simulink model "Lab3_BreakLight_replacement"  (R2026b)
settings: Solver=FixedStepAuto  StopTime=10  EnableMultiTasking=on
PreLoadFcn:
  | vehicle_data;
undefined symbols (not defined in the file or in its folder): DiscIntNeverNeededParam, magnitude, veh1, veh2, veh3
libraries: simulink x3, sldvlib x1
settings Model: DVDesignModelName=Lab3_BreakLight  STM32="{\"AnalogInput\":[{\"ID\":\"ELEC49X_Vehicle_Model:530\"},{\"ID\":\"1302\"}],\"CANWrite\":[{\"ID\":\"ELEC49X_Vehicle_Model:534\"},{\"ID\":\"ELEC49X_Vehicle_Model:535\"},{\"ID\":\"1311\"},{\"ID\":\"1312\"}],\"DigitalPortRead\":[{\"ID\":\"ELEC49X_Vehicle_Model:563\"},{\"ID\":\"ELEC49X_Vehicle_Model:564\"},{\"ID\":\"ELEC49X_Vehicle_Model:565\"},{\"ID\":\"ELEC49X_Vehicle_Model:566\"},{\"ID\":\"ELEC49X_Vehicle_Model:567\"},{\"ID\":\"ELEC49X_Vehicle_Model:589\"},{\"ID\":\"ELEC49X_Vehicle_Model:1023\"},{\"ID\":\"1368\"},{\"ID\":\"1369\"},{\"ID\":\"1370\"},{\"ID\":\"1371\"},{\"ID\":\"1372\"},{\"ID\":\"1401\"},{\"ID\":\"1402\"}],\"SPIControllerTransmit\":[{\"ID\":\"ELEC49X_Vehicle_Model:953\"},{\"ID\":\"1404\"}],\"SPIControllerReceive\":[{\"ID\":\"ELEC49X_Vehicle_Model:1097\"},{\"ID\":\"1403\"}]}"  Creator=jckwe  LastModifiedBy=balog
settings OptimizationCC: DefaultParameterBehavior=Inlined  DifferentSizesBufferReuse=on  EfficientTunableParamExpr=on  EnhancedBackFolding=on  MaxStackSize=64  OptimizationCustomize=off  OptimizeBlockOrder=speed  PassReuseOutputArgsAs=Individual arguments  RemoveInternalMemoryZeroInit=on  RemoveRootLevelIOMemoryZeroInit=on
settings DebuggingCC: ParameterTunabilityLossMsg=error  SaveWithDisabledLinksMsg=none  SaveWithParameterizedLinksMsg=none
settings HardwareCC: ProdHWDeviceType=ARM Compatible->ARM Cortex-M  ProdLargestAtomicFloat=Double  ProdLargestAtomicInteger=Long  ProdLongLongMode=on
settings SFSimCC: MATLABDynamicMemAlloc=off
settings RTWCC: BuildConfiguration=Faster Runs  Description=Embedded Coder  GPUComputeCapability=5.0  GenerateReport=on  HardwareBoard=STM32F4xx Based  SystemTargetFile=ert.tlc  TLCOptions=-aInlineSetEventsForThisBaseRateFcn=TLC_FALSE -aSuppressMultiTaskScheduler=TLC_FALSE -aRateBasedStepFcn=1  TemplateMakefile=ert_default_tmf
settings CodeAppCC: ForceParamTrailComments=on  IgnoreCustomStorageClasses=off  InsertBlockDesc=on  OperatorAnnotations=on  SFDataObjDesc=on  SimulinkDataObjDesc=on
settings ERTTargetCC: CodeReplacementLibrary=ARM Cortex-M  ExtModeIntrfLevel=Level2 - Open  ExtModeMexFile=ext_xcp  ExtModeStaticAlloc=on  SupportContinuousTime=on
settings ConfigComp: DVCodeAnalysisIgnoreVolatile=off  DVDefectChecker=on  DVDetectOutOfBounds=on  DVHarnessSource=Signal Editor  DVModelCoverageObjectives=MCDC  DVModelReferenceHarness=on  DVParametersConfigFileName=vehicle_data.m  DVSFcnSupport=off  DVTestSuiteOptimization=Auto

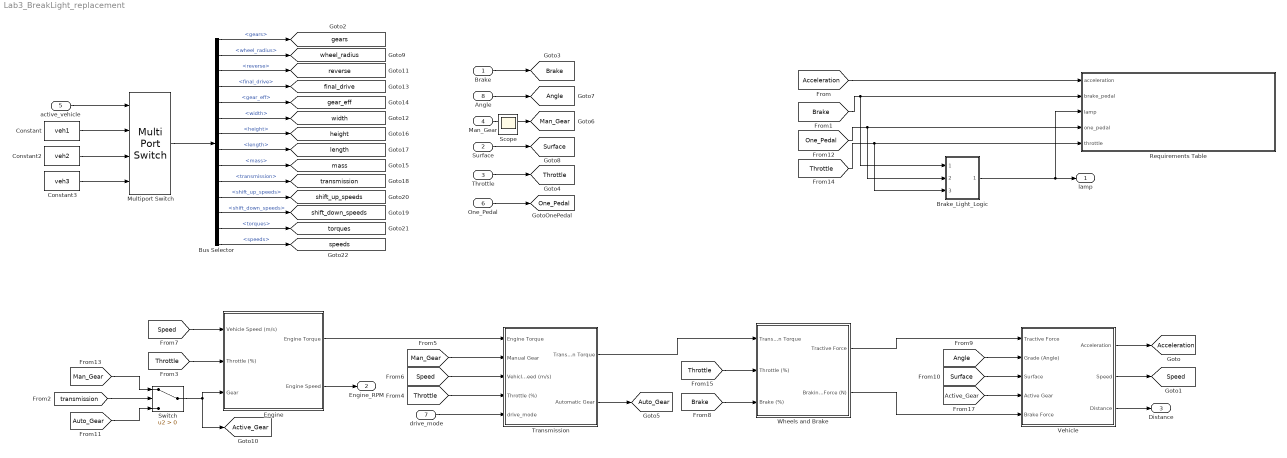
== system Lab3_BreakLight_replacement ==
  Brake : Inport
  Surface : Inport  Port=2
  Throttle : Inport  Port=3  OutMin=0  OutMax=100  OutDataTypeStr=double  LockScale=on
  Man_Gear : Inport  Port=4  OutDataTypeStr=int8
  active_vehicle : Inport  Port=5  OutMin=1  OutMax=3
  One_Pedal : Inport  Port=6  OutMin=0  OutDataTypeStr=int8
  drive_mode : Inport  Port=7  OutMin=-1  OutMax=3  OutDataTypeStr=int8
  Angle : Inport  Port=8
  Brake_Light_Logic : Subsystem
  Bus Selector : BusSelector  OutputSignals=gears,wheel_radius,reverse,final_drive,gear_eff,width,height,length,mass,transmission,shift_up_speeds,shift_down_speeds,torques,speeds
  Constant : Constant  Value=veh1  OutDataTypeStr=Bus: VehicleBus
  Constant2 : Constant  Value=veh2  OutDataTypeStr=Bus: VehicleBus
  Constant3 : Constant  Value=veh3  OutDataTypeStr=Bus: VehicleBus
  Engine : Subsystem
      mask Display: image('Engine Icon.png',[40 40 60 60]);
  Multiport Switch : MultiPortSwitch  SaturateOnIntegerOverflow=off  InputSameDT=off
  Requirements Table : Requirements Table  TreatAsAtomicUnit=on
  Switch : Switch  Criteria=u2 > Threshold  SaturateOnIntegerOverflow=off  InputSameDT=off
  Transmission : Subsystem
      mask Display: image('Transmission Icon.png', [40 40 60 60]);
  Vehicle : Subsystem
      mask Display: image('Vehicle Icon.png', [40 40 60 60]);
  Wheels and Brake : Subsystem
      mask Display: image('Wheel Icon.png', [40 40 60 60]);
  lamp : Outport
  Engine_RPM : Outport  Port=2
  Distance : Outport  Port=3
  Scope : Scope
  tag scope: Acceleration=global, Active_Gear=global, Angle=global, Auto_Gear=global, Brake=global, Man_Gear=global, One_Pedal=global, Speed=global, Surface=global, Throttle=global, final_drive=global, gear_eff=global, gears=global, height=global, length=global, mass=global, reverse=global, shift_down_speeds=global, shift_up_speeds=global, speeds=global, torques=global, transmission=global, wheel_radius=global, width=global
  wires:
  Vehicle/3(Distance) -> Distance/1
  Vehicle/2(Speed) -> [Speed]
  Vehicle/1(Acceleration) -> [Acceleration]
  Transmission/1(Transmission Torque) -> Wheels and Brake/1(Transmission Torque)
  Engine/1(Engine Torque) -> Transmission/1(Engine Torque)
  Wheels and Brake/1(Tractive Force) -> Vehicle/1(Tractive Force)
  [Throttle] -> Engine/2(Throttle (%))
  [Throttle] -> Transmission/4(Throttle (%))
  [Speed] -> Transmission/3(Vehicle Speed (m/s))
  [Speed] -> Engine/1(Vehicle Speed (m/s))
  [Brake] -> Wheels and Brake/3(Brake (%))
  [Angle] -> Vehicle/2(Grade (Angle))
  [Surface] -> Vehicle/3(Surface)
  Transmission/2(Automatic Gear) -> [Auto_Gear]
  Engine/2(Engine Speed) -> Engine_RPM/1
  Switch/1 -> [Active_Gear], Engine/3(Gear)
  [transmission] -> Switch/2
  [Man_Gear] -> Switch/1
  [Auto_Gear] -> Switch/3
  [Active_Gear] -> Vehicle/4(Active Gear)
  Wheels and Brake/2(Braking Force (N)) -> Vehicle/5(Brake Force)
  [Throttle] -> Wheels and Brake/2(Throttle (%))
  Brake/1 -> [Brake]
  Angle/1 -> [Angle]
  Man_Gear/1 -> [Man_Gear]
  Surface/1 -> [Surface]
  [Brake] -> Brake_Light_Logic/1(Brake), Requirements Table/2(brake_pedal)
  active_vehicle/1 -> Multiport Switch/1
  Constant/1 -> Multiport Switch/2
  Constant2/1 -> Multiport Switch/3
  Constant3/1 -> Multiport Switch/4
  Multiport Switch/1 -> Bus Selector/1
  Bus Selector/1 -> [gears]  "<gears>"
  Bus Selector/3 -> [reverse]  "<reverse>"
  Bus Selector/2 -> [wheel_radius]  "<wheel_radius>"
  Bus Selector/14 -> [speeds]  "<speeds>"
  Bus Selector/13 -> [torques]  "<torques>"
  Bus Selector/12 -> [shift_down_speeds]  "<shift_down_speeds>"
  Bus Selector/10 -> [transmission]  "<transmission>"
  Bus Selector/9 -> [mass]  "<mass>"
  Bus Selector/11 -> [shift_up_speeds]  "<shift_up_speeds>"
  Bus Selector/8 -> [length]  "<length>"
  Bus Selector/7 -> [height]  "<height>"
  Bus Selector/6 -> [width]  "<width>"
  Bus Selector/5 -> [gear_eff]  "<gear_eff>"
  Bus Selector/4 -> [final_drive]  "<final_drive>"
  Throttle/1 -> [Throttle]
  [Man_Gear] -> Transmission/2(Manual Gear)
  One_Pedal/1 -> [One_Pedal]
  drive_mode/1 -> Transmission/5(drive_mode)
  [Acceleration] -> Requirements Table/1(acceleration)
  [One_Pedal] -> Brake_Light_Logic/2(One_Pedal), Requirements Table/4(one_pedal)
  [Throttle] -> Brake_Light_Logic/3(Throttle), Requirements Table/5(throttle)
  Brake_Light_Logic/1(Out1) -> lamp/1, Requirements Table/3(lamp)

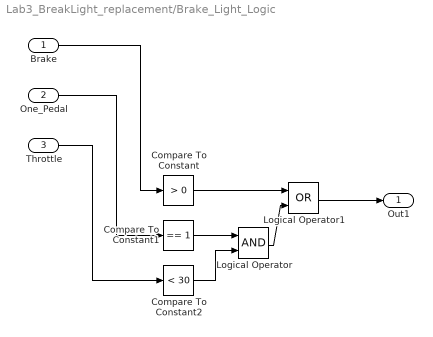
== system Lab3_BreakLight_replacement/Brake_Light_Logic ==
  Brake : Inport
  One_Pedal : Inport  Port=2
  Throttle : Inport  Port=3
  Compare To Constant : simulink/Logic and Bit Operations/Compare To Constant  relop=>  const=0  OutDataTypeStr=boolean
  Compare To Constant1 : simulink/Logic and Bit Operations/Compare To Constant  relop===  const=1  OutDataTypeStr=boolean
  Compare To Constant2 : simulink/Logic and Bit Operations/Compare To Constant  relop=<  const=30  OutDataTypeStr=boolean
  Logical Operator : Logic  AllPortsSameDT=off  OutDataTypeStr=boolean
  Logical Operator1 : Logic  Operator=OR  AllPortsSameDT=off  OutDataTypeStr=boolean
  Out1 : Outport
  wires:
  Logical Operator1/1 -> Out1/1
  Logical Operator/1 -> Logical Operator1/2
  Brake/1 -> Compare To Constant/1
  Throttle/1 -> Compare To Constant2/1
  Compare To Constant2/1 -> Logical Operator/2
  One_Pedal/1 -> Compare To Constant1/1
  Compare To Constant/1 -> Logical Operator1/1
  Compare To Constant1/1 -> Logical Operator/1

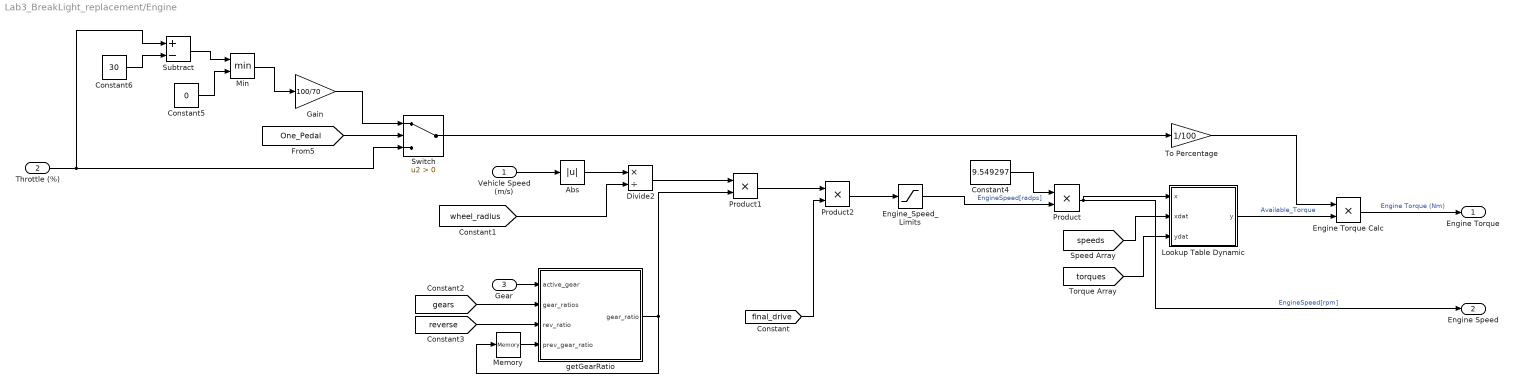
== system Lab3_BreakLight_replacement/Engine ==
  Vehicle Speed (m/s) : Inport
  Throttle (%) : Inport  Port=2
  Gear : Inport  Port=3  OutDataTypeStr=int8
  Abs : Abs  SaturateOnIntegerOverflow=off
  Constant4 : Constant  Value=9.549297
  Constant5 : Constant  Value=0
  Constant6 : Constant  Value=30
  Divide2 : Product  Inputs=*/
  Engine Torque Calc : Product
  Engine_Speed_Limits : Saturate  UpperLimit=800  LowerLimit=80
  Gain : Gain  Gain=100/70
  Lookup Table Dynamic : Subsystem  mask(Sldv Lookup Table Dynamic Replacement){LookUpMeth=Interpolation-Use End Values, OutDataTypeStr=double, LockScale=off, RndMeth=Floor, DoSatur=off}
      mask prompts: LookUpMeth "Lookup Method:"; OutDataTypeStr "Output data type:"; LockScale "Lock output data type setting against changes by the fixed-point tools"; RndMeth "Integer rounding mode:"; DoSatur "Do Saturation"
      mask init:
      | mode = LookUpMeth-1;
      mask TypeOptions LookUpMeth: Interpolation-Extrapolation | Interpolation-Use End Values | Use Input Nearest | Use Input Below | Use Input Above
      mask Callback OutDataTypeStr: fixptdialog(gcbh)
      mask TypeOptions RndMeth: Ceiling | Convergent | Floor | Nearest | Round | Simplest | Zero
  Memory : Memory
  Min : MinMax  Inputs=2
  Product : Product
  Product1 : Product
  Product2 : Product
  Subtract : Sum  Inputs=+-
  Switch : Switch  Criteria=u2 > Threshold  SaturateOnIntegerOverflow=off  InputSameDT=off
  To Percentage : Gain  Gain=1/100
  getGearRatio : MATLAB Function  TreatAsAtomicUnit=on
  Engine Torque : Outport
  Engine Speed : Outport  Port=2
  wires:
  To Percentage/1 -> Engine Torque Calc/1
  Engine_Speed_Limits/1 -> Product/2  "EngineSpeed[radps]"
  Product/1 -> Lookup Table Dynamic/1(x), Engine Speed/1  "EngineSpeed[rpm]"
  [speeds] -> Lookup Table Dynamic/2(xdat)
  [torques] -> Lookup Table Dynamic/3(ydat)
  Engine Torque Calc/1 -> Engine Torque/1  "Engine Torque (Nm)"
  Gear/1 -> getGearRatio/1(active_gear)
  [wheel_radius] -> Divide2/2
  Vehicle Speed (m/s)/1 -> Abs/1
  Divide2/1 -> Product1/1
  getGearRatio/1(gear_ratio) -> Product1/2, Memory/1
  [gears] -> getGearRatio/2(gear_ratios)
  [reverse] -> getGearRatio/3(rev_ratio)
  Memory/1 -> getGearRatio/4(prev_gear_ratio)
  Constant4/1 -> Product/1
  Product1/1 -> Product2/1
  [final_drive] -> Product2/2
  Product2/1 -> Engine_Speed_Limits/1
  Abs/1 -> Divide2/1
  [One_Pedal] -> Switch/2
  Switch/1 -> To Percentage/1
  Throttle (%)/1 -> Subtract/1, Switch/3
  Gain/1 -> Switch/1
  Constant6/1 -> Subtract/2
  Subtract/1 -> Min/1
  Min/1 -> Gain/1
  Constant5/1 -> Min/2
  Lookup Table Dynamic/1(y) -> Engine Torque Calc/2  "Available_Torque"

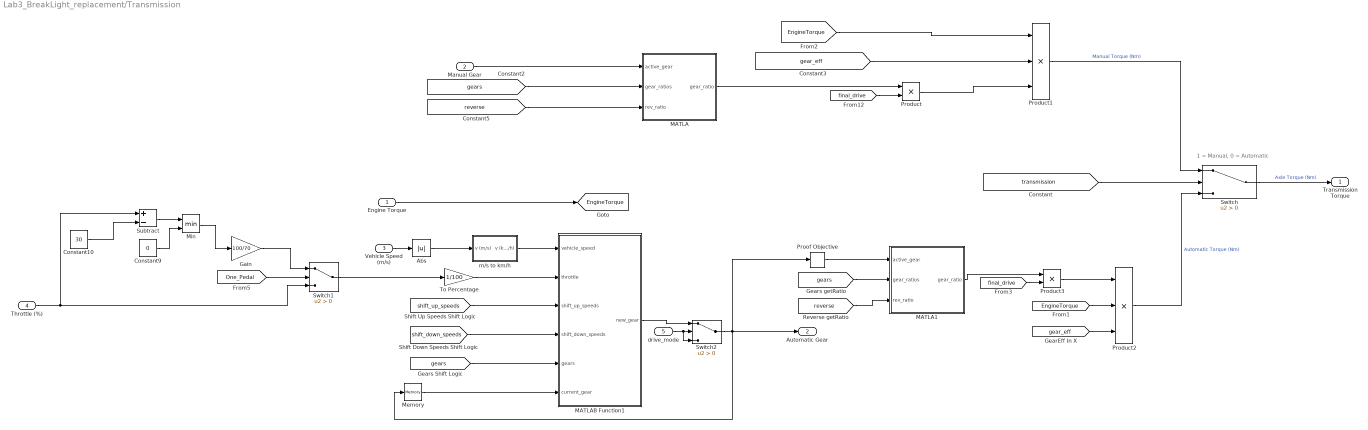
== system Lab3_BreakLight_replacement/Transmission ==
  note: 1 = Manual, 0 = Automatic
  Engine Torque : Inport
  Manual Gear : Inport  Port=2  OutDataTypeStr=int8
  Vehicle Speed (m/s) : Inport  Port=3
  Throttle (%) : Inport  Port=4
  drive_mode : Inport  Port=5  OutMin=-1  OutMax=127  OutDataTypeStr=int8
  Abs : Abs  SaturateOnIntegerOverflow=off
  Constant10 : Constant  Value=30
  Constant9 : Constant  Value=0
  Gain : Gain  Gain=100/70
  MATLA : MATLAB Function  TreatAsAtomicUnit=on
  MATLA1 : MATLAB Function  TreatAsAtomicUnit=on
  MATLAB Function1 : MATLAB Function  TreatAsAtomicUnit=on
  Memory : Memory
  Min : MinMax  Inputs=2
  Product : Product
  Product1 : Product  Inputs=3
  Product2 : Product  Inputs=3
  Product3 : Product
  Proof Objective : sldvlib/Objectives and Constraints/Proof Objective  enabled=on  customAVTBlockType=Proof Objective  intervals={-1, 127}  dispValues=on  outEnabled=on  enableStopSim=off
      settings: AttributesFormatString=%<intervals>
  Subtract : Sum  Inputs=+-
  Switch : Switch  Criteria=u2 > Threshold  SaturateOnIntegerOverflow=off  InputSameDT=off
  Switch1 : Switch  Criteria=u2 > Threshold  SaturateOnIntegerOverflow=off  InputSameDT=off
  Switch2 : Switch  Criteria=u2 > Threshold  SaturateOnIntegerOverflow=off  InputSameDT=off
  To Percentage : Gain  Gain=1/100
  m/s to km/h : Subsystem
  Transmission Torque : Outport
  Automatic Gear : Outport  Port=2
  tag scope: EngineTorque=global
  wires:
  [transmission] -> Switch/2
  MATLA/1(gear_ratio) -> Product/1
  Manual Gear/1 -> MATLA/1(active_gear)
  [gear_eff] -> Product1/2
  Engine Torque/1 -> [EngineTorque]
  [EngineTorque] -> Product1/1
  Product1/1 -> Switch/1  "Manual Torque (Nm)"
  Switch1/1 -> To Percentage/1
  Vehicle Speed (m/s)/1 -> Abs/1
  MATLA1/1(gear_ratio) -> Product3/1
  [EngineTorque] -> Product2/2
  [gear_eff] -> Product2/3
  Product2/1 -> Switch/3  "Automatic Torque (Nm)"
  m/s to km/h/1(v (km/h)) -> MATLAB Function1/1(vehicle_speed)
  Switch/1 -> Transmission Torque/1  "Axle Torque (Nm)"
  [gears] -> MATLA/2(gear_ratios)
  [gears] -> MATLA1/2(gear_ratios)
  [shift_up_speeds] -> MATLAB Function1/3(shift_up_speeds)
  [shift_down_speeds] -> MATLAB Function1/4(shift_down_speeds)
  [gears] -> MATLAB Function1/5(gears)
  Memory/1 -> MATLAB Function1/6(current_gear)
  [reverse] -> MATLA/3(rev_ratio)
  [reverse] -> MATLA1/3(rev_ratio)
  Abs/1 -> m/s to km/h/1(v (m/s))
  To Percentage/1 -> MATLAB Function1/2(throttle)
  Constant9/1 -> Min/2
  Gain/1 -> Switch1/1
  Min/1 -> Gain/1
  [One_Pedal] -> Switch1/2
  Constant10/1 -> Subtract/2
  Throttle (%)/1 -> Subtract/1, Switch1/3
  Subtract/1 -> Min/1
  Proof Objective/1 -> MATLA1/1(active_gear)
  drive_mode/1 -> Switch2/3, Switch2/2
  MATLAB Function1/1(new_gear) -> Switch2/1
  Switch2/1 -> Memory/1, Proof Objective/1, Automatic Gear/1
  [final_drive] -> Product/2
  Product/1 -> Product1/3
  [final_drive] -> Product3/2
  Product3/1 -> Product2/1

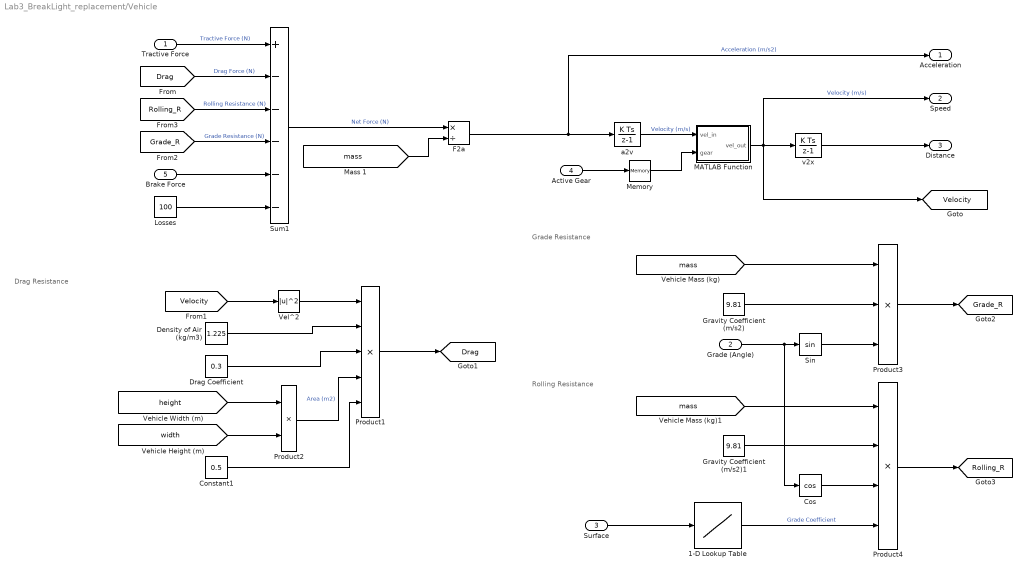
== system Lab3_BreakLight_replacement/Vehicle ==
  note: Rolling Resistance
  note: Grade Resistance
  note: Drag Resistance
  Tractive Force : Inport
  Grade (Angle) : Inport  Port=2
  Surface : Inport  Port=3
  Active Gear : Inport  Port=4
  Brake Force : Inport  Port=5
  1-D Lookup Table : Lookup_n-D  NumberOfTableDimensions=1  BreakpointsForDimension1=[0:4]  Table=[0.015, 0.025, 0.045, 0.09, 0.12]  InternalRulePriority=Speed  RndMeth=Simplest
  Constant1 : Constant  Value=0.5
  Cos : Trigonometry  Operator=cos
  Density of Air (kg/m3) : Constant  Value=1.225
  Drag Coefficient : Constant  Value=0.3
  F2a : Product  Inputs=*/
  Gravity Coefficient (m/s2) : Constant  Value=9.81
  Gravity Coefficient (m/s2)1 : Constant  Value=9.81
  Losses : Constant  Value=100
  MATLAB Function : MATLAB Function  TreatAsAtomicUnit=on
  Memory : Memory
  Product1 : Product  Inputs=5
  Product2 : Product
  Product3 : Product  Inputs=3
  Product4 : Product  Inputs=4
  Sin : Trigonometry
  Sum1 : Sum  Inputs=+-----
  Vel^2 : Math  Operator=magnitude^2  SignedPower=on
  a2v : DiscreteIntegrator  SampleTime=-1  LimitOutput=on  UpperSaturationLimit=100  LowerSaturationLimit=0  ICPrevOutput=DiscIntNeverNeededParam  ICPrevScaledInput=DiscIntNeverNeededParam
  v2x : DiscreteIntegrator  SampleTime=-1  ICPrevOutput=DiscIntNeverNeededParam  ICPrevScaledInput=DiscIntNeverNeededParam
  Acceleration : Outport
  Speed : Outport  Port=2
  Distance : Outport  Port=3
  tag scope: Drag=global, Grade_R=global, Rolling_R=global, Velocity=global
  wires:
  Tractive Force/1 -> Sum1/1  "Tractive Force (N)"
  [Drag] -> Sum1/2  "Drag Force (N)"
  [Rolling_R] -> Sum1/3  "Rolling Resistance (N)"
  [Grade_R] -> Sum1/4  "Grade Resistance (N)"
  Sum1/1 -> F2a/1  "Net Force (N)"
  [mass] -> F2a/2
  [Velocity] -> Vel^2/1
  Vel^2/1 -> Product1/1
  [height] -> Product2/1
  [width] -> Product2/2
  Product2/1 -> Product1/4  "Area (m2)"
  Density of Air (kg/m3)/1 -> Product1/2
  Drag Coefficient/1 -> Product1/3
  Product1/1 -> [Drag]
  [mass] -> Product3/1
  Gravity Coefficient (m/s2)/1 -> Product3/2
  Sin/1 -> Product3/3
  Grade (Angle)/1 -> Cos/1, Sin/1
  Product3/1 -> [Grade_R]
  Cos/1 -> Product4/3
  [mass] -> Product4/1
  Product4/1 -> [Rolling_R]
  Gravity Coefficient (m/s2)1/1 -> Product4/2
  Surface/1 -> 1-D Lookup Table/1
  1-D Lookup Table/1 -> Product4/4  "Grade Coefficient"
  F2a/1 -> Acceleration/1, a2v/1  "Acceleration (m/s2)"
  MATLAB Function/1(vel_out) -> v2x/1, Speed/1, [Velocity]  "Velocity (m/s)"
  Brake Force/1 -> Sum1/5
  Constant1/1 -> Product1/5
  a2v/1 -> MATLAB Function/1(vel_in)  "Velocity (m/s)"
  Active Gear/1 -> Memory/1
  Memory/1 -> MATLAB Function/2(gear)
  Losses/1 -> Sum1/6
  v2x/1 -> Distance/1

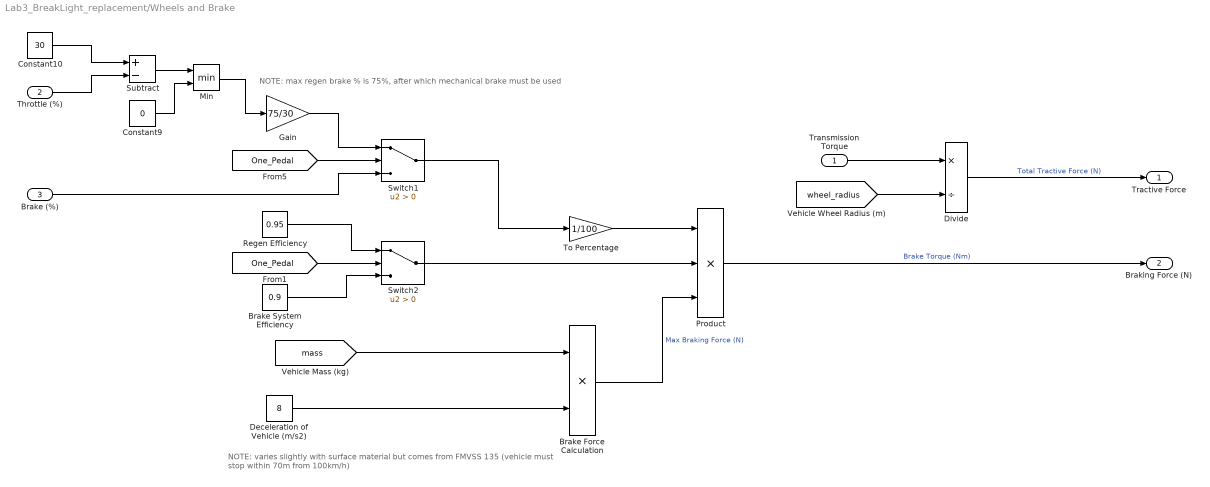
== system Lab3_BreakLight_replacement/Wheels and Brake ==
  note: NOTE: varies slightly with surface material but comes from FMVSS 135 (vehicle
      | must stop within 70m from 100km/h)
  note: NOTE: max regen brake % is 75%, after which mechanical brake must be used
  Transmission Torque : Inport
  Throttle (%) : Inport  Port=2
  Brake (%) : Inport  Port=3
  Brake Force Calculation : Product
  Brake System Efficiency : Constant  Value=0.9
  Constant10 : Constant  Value=30
  Constant9 : Constant  Value=0
  Deceleration of Vehicle (m/s2) : Constant  Value=8
  Divide : Product  Inputs=*/
  Gain : Gain  Gain=75/30
  Min : MinMax  Inputs=2
  Product : Product  Inputs=3
  Regen Efficiency : Constant  Value=0.95
  Subtract : Sum  Inputs=+-
  Switch1 : Switch  Criteria=u2 > Threshold  SaturateOnIntegerOverflow=off  InputSameDT=off
  Switch2 : Switch  Criteria=u2 > Threshold  SaturateOnIntegerOverflow=off  InputSameDT=off
  To Percentage : Gain  Gain=1/100
  Tractive Force : Outport
  Braking Force (N) : Outport  Port=2
  wires:
  Switch2/1 -> Product/2
  Switch1/1 -> To Percentage/1
  Brake Force Calculation/1 -> Product/3  "Max Braking Force (N)"
  Deceleration of Vehicle (m/s2)/1 -> Brake Force Calculation/2
  [mass] -> Brake Force Calculation/1
  Transmission Torque/1 -> Divide/1
  Divide/1 -> Tractive Force/1  "Total Tractive Force (N)"
  To Percentage/1 -> Product/1
  [wheel_radius] -> Divide/2
  Product/1 -> Braking Force (N)/1  "Brake Torque (Nm)"
  Subtract/1 -> Min/1
  Constant9/1 -> Min/2
  Min/1 -> Gain/1
  [One_Pedal] -> Switch1/2
  Gain/1 -> Switch1/1
  Brake (%)/1 -> Switch1/3
  [One_Pedal] -> Switch2/2
  Brake System Efficiency/1 -> Switch2/3
  Regen Efficiency/1 -> Switch2/1
  Constant10/1 -> Subtract/1
  Throttle (%)/1 -> Subtract/2

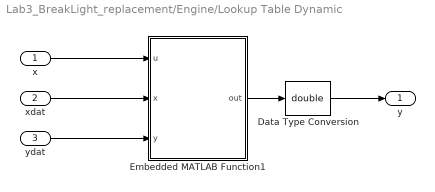
== system Lab3_BreakLight_replacement/Engine/Lookup Table Dynamic ==
  x : Inport  OutDataTypeStr=double  PortDimensions=1
  xdat : Inport  Port=2  OutDataTypeStr=double  PortDimensions=[1 21]
  ydat : Inport  Port=3  OutDataTypeStr=double  PortDimensions=[1 21]
  Data Type Conversion : DataTypeConversion  OutDataTypeStr=double  SaturateOnIntegerOverflow=off  RndMeth=Floor
  Embedded MATLAB Function1 : MATLAB Function  DisableCoverage=on  TreatAsAtomicUnit=on
  y : Outport  OutDataTypeStr=double  PortDimensions=1
  wires:
  Embedded MATLAB Function1/1(out) -> Data Type Conversion/1
  ydat/1 -> Embedded MATLAB Function1/3(y)
  xdat/1 -> Embedded MATLAB Function1/2(x)
  x/1 -> Embedded MATLAB Function1/1(u)
  Data Type Conversion/1 -> y/1

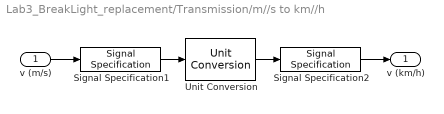
== system Lab3_BreakLight_replacement/Transmission/m//s to km//h ==
  v (m/s) : Inport
  Signal Specification1 : SignalSpecification  Unit=m/s
  Signal Specification2 : SignalSpecification  Unit=km/hr
  Unit Conversion : UnitConversion
  v (km/h) : Outport
  wires:
  v (m/s)/1 -> Signal Specification1/1
  Unit Conversion/1 -> Signal Specification2/1
  Signal Specification1/1 -> Unit Conversion/1
  Signal Specification2/1 -> v (km/h)/1

== matlab function Lab3_BreakLight_replacement/Transmission/MATLA ==
  data: active_gear input; gear_ratio output; gear_ratios input; rev_ratio input
function gear_ratio = getGearRatio(active_gear, gear_ratios, rev_ratio)  
    num_gears = sum(gear_ratios > 0);

    % Return the selected gear ratio
    if (active_gear == -1) 
        gear_ratio = rev_ratio;
    elseif (active_gear == 0)
        gear_ratio = 0; 
    elseif (active_gear <= num_gears)
        gear_ratio = gear_ratios(active_gear);
    else
        gear_ratio = 0;
    end
end

== matlab function Lab3_BreakLight_replacement/Transmission/MATLAB Function1 ==
  data: vehicle_speed input; new_gear output; throttle input; shift_up_speeds input; shift_down_speeds input; gears input; current_gear input int8
function new_gear = gearShiftLogic(vehicle_speed, throttle, shift_up_speeds, shift_down_speeds, gears, current_gear)
    num_gears = sum(gears > 0);
   
    if current_gear == 0
        current_gear = int8(1); % Default to first gear
    end
    
    % Define throttle levels (0% throttle, 50%, 100%)
    throttle_levels = [0, 0.5, 1];
    
    % Interpolate shift speeds based on throttle level for the selected vehicle
    up_th = interp1(throttle_levels, shift_up_speeds, throttle, 'linear', 'extrap');
    down_th = interp1(throttle_levels, shift_down_speeds, throttle, 'linear', 'extrap');

    % Ensure that up_th and down_th are scalars (if necessary, use indexing)
    up_th = up_th(current_gear);  % Get the specific threshold for the current gear
    down_th = down_th(current_gear);  % Get the specific threshold for the current gear

    % Upshift if speed exceeds threshold and current gear is not the max gear
    if vehicle_speed > up_th && current_gear < num_gears
        current_gear = current_gear + 1;
    end

    % Downshift if speed drops below threshold and current gear is not the min gear
    if vehicle_speed < down_th && current_gear > 1
        current_gear = current_gear - 1;
    end

    % Output the new gear
    new_gear = current_gear;
end

== matlab function Lab3_BreakLight_replacement/Transmission/MATLA1 ==
  data: active_gear input; gear_ratio output; gear_ratios input; rev_ratio input
function gear_ratio = getGearRatio(active_gear, gear_ratios, rev_ratio)
    num_gears = sum(gear_ratios > 0);
    % Return the selected gear ratio
    if (active_gear == -1) 
        gear_ratio = rev_ratio;
    elseif (active_gear == 0)
        gear_ratio = 0; 
    elseif (active_gear <= num_gears)
        gear_ratio = gear_ratios(active_gear);
    else
        gear_ratio = 0;
    end
end

== matlab function Lab3_BreakLight_replacement/Engine/getGearRatio ==
  data: active_gear input; gear_ratio output; gear_ratios input; rev_ratio input; prev_gear_ratio input
function gear_ratio = getGearRatio(active_gear, gear_ratios, rev_ratio, prev_gear_ratio) 
    if (prev_gear_ratio == 0) 
        prev_gear_ratio = gear_ratios(1); % default to first
    end
    if (active_gear == -1) 
        gear_ratio = rev_ratio;
    elseif (active_gear == 0)
        gear_ratio = prev_gear_ratio; 
    elseif (active_gear <= length(gear_ratios))
        gear_ratio = gear_ratios(active_gear);
    else
        gear_ratio = prev_gear_ratio;
    end
end

== matlab function Lab3_BreakLight_replacement/Vehicle/MATLAB Function ==
  data: vel_in input; gear input; vel_out output
function vel_out = vel_function(vel_in, gear)
    if gear == -1
        vel_out = -vel_in;
    else
        vel_out = vel_in;
    end
end

== stateflow chart Lab3_BreakLight_replacement/Requirements Table ==
  (default) -> (junction 1073742409)
  (junction 1073742409) -> (junction 1073742410) : {
      | % SF_REQ_REV_09
      | }
  (junction 1073742410) -> (junction 1073742412) : {
      | % ExcEvals:
      | % PriEvals:
      | }
  (junction 1073742412) -> (junction 1073742414) : {
      | % HEADER_ASSIGNMENTS
      |
      | }
  (junction 1073742414) -> (junction 1073742416) : {
      | % START_A_4
      | }
  (junction 1073742416) -> (junction 1073742418) : {
      | }
  (junction 1073742418) -> (junction 1073742420) : {
      | reqtable_assumption((brake_pedal >= 0 && brake_pedal <= 100), 4);
      | }
  (junction 1073742420) -> (junction 1073742422) : {
      | }
  (junction 1073742422) -> (junction 1073742424) : {
      | % END_A_4
      | }
  (junction 1073742424) -> (junction 1073742426) : {
      | % START_A_25
      | }
  (junction 1073742426) -> (junction 1073742428) : {
      | }
  (junction 1073742428) -> (junction 1073742430) : {
      | reqtable_assumption((throttle >= 0 && throttle <= 100), 25);
      | }
  (junction 1073742430) -> (junction 1073742432) : {
      | }
  (junction 1073742432) -> (junction 1073742434) : {
      | % END_A_25
      | }
  (junction 1073742434) -> (junction 1073742436) : {
      | % START_A_28
      | }
  (junction 1073742436) -> (junction 1073742438) : {
      | }
  (junction 1073742438) -> (junction 1073742440) : {
      | reqtable_assumption((one_pedal == 0 || one_pedal == 1), 28);
      | }
  (junction 1073742440) -> (junction 1073742442) : {
      | }
  (junction 1073742442) -> (junction 1073742444) : {
      | % END_A_28
      | }
  (junction 1073742444) -> (junction 1073742446) : {
      | % START_R_1
      | }
  (junction 1073742446) -> (junction 1073742448) : {
      | }
  (junction 1073742448) -> (junction 1073742450)
  (junction 1073742450) -> (junction 1073742452) [order 1] : [(brake_pedal > 0)]
  (junction 1073742450) -> (junction 1073742458) [order 2]
  (junction 1073742452) -> (junction 1073742454) : {
      | reqtable_postcondition((lamp == true), 'R:1');
      |
      |
      | }
  (junction 1073742454) -> (junction 1073742456) : {
      | }
  (junction 1073742456) -> (junction 1073742458)
  (junction 1073742458) -> (junction 1073742460)
  (junction 1073742460) -> (junction 1073742462) : {
      | % END_R_1
      | }
  (junction 1073742462) -> (junction 1073742464) : {
      | % START_R_13
      | }
  (junction 1073742464) -> (junction 1073742466) : {
      | }
  (junction 1073742466) -> (junction 1073742468)
  (junction 1073742468) -> (junction 1073742470) [order 1] : [(one_pedal == 1 && throttle < 30)]
  (junction 1073742468) -> (junction 1073742476) [order 2]
  (junction 1073742470) -> (junction 1073742472) : {
      | reqtable_postcondition((lamp == true), 'R:2');
      |
      |
      | }
  (junction 1073742472) -> (junction 1073742474) : {
      | }
  (junction 1073742474) -> (junction 1073742476)
  (junction 1073742476) -> (junction 1073742478)
  (junction 1073742478) -> (junction 1073742480) : {
      | % END_R_13
      | }
  (junction 1073742480) -> (junction 1073742482) : {
      | % START_R_16
      | }
  (junction 1073742482) -> (junction 1073742484) : {
      | }
  (junction 1073742484) -> (junction 1073742486)
  (junction 1073742486) -> (junction 1073742488) [order 1] : [(brake_pedal <= 0 && ~(one_pedal == 1 && throttle < 30))]
  (junction 1073742486) -> (junction 1073742494) [order 2]
  (junction 1073742488) -> (junction 1073742490) : {
      | reqtable_postcondition((lamp == false), 'R:3');
      |
      |
      | }
  (junction 1073742490) -> (junction 1073742492) : {
      | }
  (junction 1073742492) -> (junction 1073742494)
  (junction 1073742494) -> (junction 1073742496)
  (junction 1073742496) -> (junction 1073742498) : {
      | % END_R_16
      | }
  (junction 1073742498) -> (junction 1073742500) : {
      | % START_R_19
      | }
  (junction 1073742500) -> (junction 1073742502) : {
      | }
  (junction 1073742502) -> (junction 1073742504) : {
      |
      |
      | }
  (junction 1073742504) -> (junction 1073742506) : {
      | }
  (junction 1073742506) -> (junction 1073742508) : {
      | % END_R_19
      | }
  (junction 1073742508) -> (junction 1073742510) : {
      | % START_R_22
      | }
  (junction 1073742510) -> (junction 1073742512) : {
      | }
  (junction 1073742512) -> (junction 1073742514) : {
      |
      |
      | }
  (junction 1073742514) -> (junction 1073742516) : {
      | }
  (junction 1073742516) -> (junction 1073742518) : {
      | % END_R_22
      | }
  data: acceleration input; brake_pedal input; lamp input; one_pedal input; throttle input

== matlab function Lab3_BreakLight_replacement/Engine/Lookup Table Dynamic/Embedded MATLAB Function1 ==
  data: u input; out output; mode parameter; x input; y input
function out = fcn(u, mode, x, y)
%#eml

% mode : Type of the lookup table
%        0 for Interpolation-Extrapolation
%        1 for Interpolation-Use End Values
%        2 for Use Input Nearest
%        3 for Use Input Below
%        4 for Use Input Above

    n = numel(x);
    inputsize = size(u);
    out = zeros(inputsize);
    inputelems = prod(inputsize);
    for idx=1:inputelems
        out(idx) = lookup_dynamic(u(idx), mode, x, y, n);
    end
end

function out = lookup_dynamic(u, mode, x, y, n)
    if mode==0
        idx = lookup_util_index_extrap(u, n, x);
        num = y(idx+1) - y(idx);
        den = x(idx+1) - x(idx);
        m = num/den;
        out = y(idx) + (m*(u-x(idx)));  
    else
        if mode==1
            if u <= x(1)                                
                idxLeft = int32(1);                                                
                out = y(idxLeft);
            elseif u >= x(n)                                                
                idxLeft = int32(n);
                out = y(idxLeft);
            else
                [idxLeft, idxRight] = lookup_util_index_no_extrap_mode1(u, n, x);
                out = lookup_util_interpolate(u, x(idxLeft), x(idxRight), ...
                    y(idxLeft), y(idxRight));
            end                        
        else
            [idxLeft, idxRight] = lookup_util_index_no_extrap(u, mode, n, x);
            switch  mode                                     
                case 2            
                    diffLeft = u - x(idxLeft);
                    diffRight = x(idxRight)-u;
                    if diffRight <= diffLeft
                        idxLeft = idxRight;
                    end
                    out = y(idxLeft);
                case 3            
                    out = y(idxLeft);
                case 4            
                    out = y(idxRight);        
            end    
        end                                                        
    end
end

function idx = lookup_util_index_extrap(u, n, x)
    idxLow = int32(1);
    idxHi = int32(n-1);   
    found = false;

    idx = idxLow;
    if u >= x(n)
        idx = idxHi;
    elseif u <= x(1)
        idx = idxLow;            
    else           
        if u<0
            for i=2:n
                if ~found && u < x(i) 
                    idx = int32(i-1);
                    found = true;
                end
            end
        else
            for i=2:n
                if ~found && u <= x(i) 
                    idx = int32(i-1);
                    found = true;
                end
            end
        end
    end         
end

function [idxLeft, idxRight] = lookup_util_index_no_extrap_mode1(u, n, x)    
    idxLow = int32(1);
    idxHi = int32(n);
    found = false;
    
    idxLeft = idxLow;
    idxRight = idxHi;       
                   
    for i=2:n
        if ~found && u < x(i)
            idxRight = int32(i);
            idxLeft = int32(i-1);
            found = true;
        end
    end            
end

function [idxLeft, idxRight] = lookup_util_index_no_extrap(u, mode, n, x)    
    idxLow = int32(1);
    idxHi = int32(n);
    found = false;
    
    idxLeft = idxLow;
    idxRight = idxHi;       
    
    if mode==4                
        if u <= x(1)
            idxRight = idxLow;
        elseif u >= x(n)
            idxLeft = idxHi;
        else        
            for i=2:n
                if ~found && u <= x(i)
                    idxRight = int32(i);
                    idxLeft = int32(i-1);
                    found = true;
                end
            end        
        end         
    else        
        if u <= x(1)
            idxRight = idxLow;
        elseif u >= x(n)
            idxLeft = idxHi;
        else        
            for i=2:n
                if ~found && u < x(i)
                    idxRight = int32(i);
                    idxLeft = int32(i-1);
                    found = true;
                end
            end        
        end         
    end           
end

function out = lookup_util_interpolate(u, xL, xR, yL, yR)
    if strcmp(class(xL),class(yL))
        if u > xL                          
            den = xR - xL;
            num = u - xL;
            ydiff = yR-yL;
            bigProd = ydiff*num;            
            ydiff = bigProd/den;
            out = yL + ydiff;  
        else
            out = yL;
        end
    else
        if isfloat(yL)
            if u > xL  
                den = double(xR - xL);
                num = double(u - xL);
                ydiff = double(yR-yL);
                bigProd = ydiff*num;                
                ydiff = bigProd/den;            
                out = yL + cast(ydiff,class(yL));  
            else
                out = yL;
            end
        else        
            if u > xL  
                den = int32(xR - xL);
                num = int32(u - xL);
                ydiff = int32(yR-yL);
                bigProd = ydiff*num;                
                ydiff = bigProd/den;            
                out = yL + cast(ydiff,class(yL));  
            else
                out = yL;
            end
        end
    end        
end
